simulink model "sim_tanque_teste"  (Simulink 8.8)
settings: Solver=ode15s  StartTime=0.0  StopTime=100  RelTol=1e-3  EnableMultiTasking=on
InitFcn:
  | sim_simb
values from neighbouring files (symbols this model uses):
  Fi_nom = 10    [sim_simb.m]
  L_nom = 2.0408    [sim_simb.m]
  T_nom = 45.4    [sim_simb.m]
  Ts = .1    (= 0.1)    [estimacao.m]    (also in sim_simb.m)
settings Model: Creator=marcio  LastModifiedBy=marcio
settings OptimizationCC: ExpressionDepthLimit=2147483647
settings ConfigComp: CovSFcnEnable=off

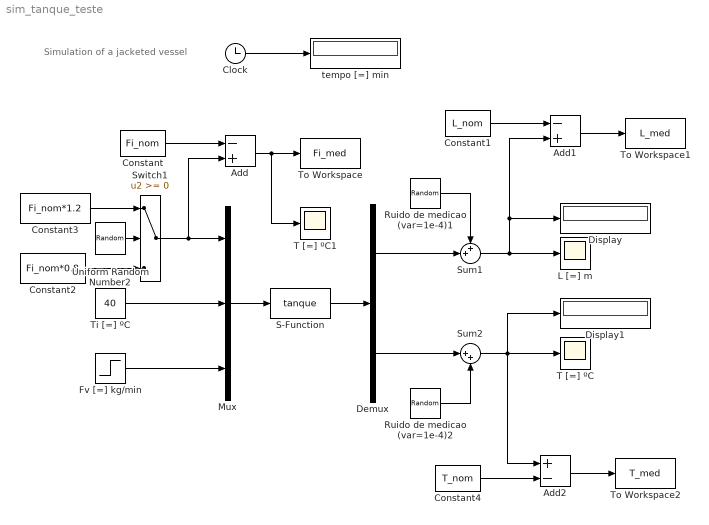
== system sim_tanque_teste ==
  note: Simulation of a jacketed vessel
  Add : Sum  Inputs=-+
  Add1 : Sum  Inputs=-+
  Add2 : Sum  Inputs=+-
  Clock : Clock
  Constant : Constant  Value=Fi_nom
  Constant1 : Constant  Value=L_nom
  Constant2 : Constant  Value=Fi_nom*0.8
  Constant3 : Constant  Value=Fi_nom*1.2
  Constant4 : Constant  Value=T_nom
  Demux : Demux  Outputs=2
  Display : Display
  Display1 : Display
  Fv [=] kg/min : Step  Time=20  Before=10  After=10  SampleTime=0
  L [=] m : Scope
  Mux : Mux  Inputs=3
  Ruido de medicao (var=1e-4)1 : RandomNumber  Variance=1e-3  Seed=78960  SampleTime=.1
  Ruido de medicao (var=1e-4)2 : RandomNumber  Variance=1e-3  Seed=78960  SampleTime=.1
  S-Function : S-Function  FunctionName=tanque  Parameters=rho,Cp,A,k,lambda  SFunctionDeploymentMode=off  EnableBusSupport=off  mask{rho=1e3, Cp=4.18, A=pi*0.5^2, k=7, lambda=2.257e4}
      mask prompts: rho "massa especifica [=] kg/m3"; Cp "calor especifico [=] kJ/kg.ºC"; A "area transversal [=] m2"; k "constante da valvula [=] m^2.5/min"; lambda "calor de vaporizacao [=] kJ/kg"
  Sum1 : Sum  Inputs=++|  SampleTime=0.1
  Sum2 : Sum  Inputs=|++  SampleTime=0.1
  Switch1 : Switch
  T [=] ºC : Scope
  T [=] ºC1 : Scope
  Ti [=] ºC : Constant  Value=40
  To Workspace : ToWorkspace  VariableName=Fi_med  SampleTime=0.1
  To Workspace1 : ToWorkspace  VariableName=L_med  SampleTime=0.1
  To Workspace2 : ToWorkspace  VariableName=T_med  SampleTime=0.1
  Uniform Random Number2 : UniformRandomNumber  SampleTime=Ts*4
  tempo [=] min : Display
  wires:
  Mux/1 -> S-Function/1
  S-Function/1 -> Demux/1
  Ti [=] ºC/1 -> Mux/2
  Fv [=] kg/min/1 -> Mux/3
  Clock/1 -> tempo [=] min/1
  Uniform Random Number2/1 -> Switch1/2
  Constant2/1 -> Switch1/3
  Constant3/1 -> Switch1/1
  Switch1/1 -> Add/2, Mux/1
  Demux/1 -> Sum1/2
  Sum1/1 -> Add1/2, Display/1, L [=] m/1
  Ruido de medicao (var=1e-4)1/1 -> Sum1/1
  Demux/2 -> Sum2/1
  Ruido de medicao (var=1e-4)2/1 -> Sum2/2
  Sum2/1 -> Add2/1, Display1/1, T [=] ºC/1
  Constant/1 -> Add/1
  Add/1 -> T [=] ºC1/1, To Workspace/1
  Constant1/1 -> Add1/1
  Add1/1 -> To Workspace1/1
  Add2/1 -> To Workspace2/1
  Constant4/1 -> Add2/2
